simulink model "FMCW_Fixedpoint_model"  (R2025b)
settings: Solver=VariableStepAuto  StartTime=0.0  StopTime=10.0  RelTol=1e-3
libraries: phaseddetectlib x1, dspsrcs4 x1, dspxfrm3 x1, dspsigops x1, dspfdesign x1
settings Model: Creator=Yahin  LastModifiedBy=Yahin

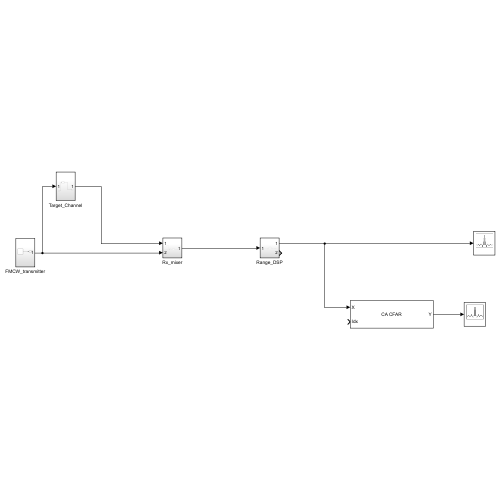
[thumbnail: Simulink's stored preview of the top-level diagram]
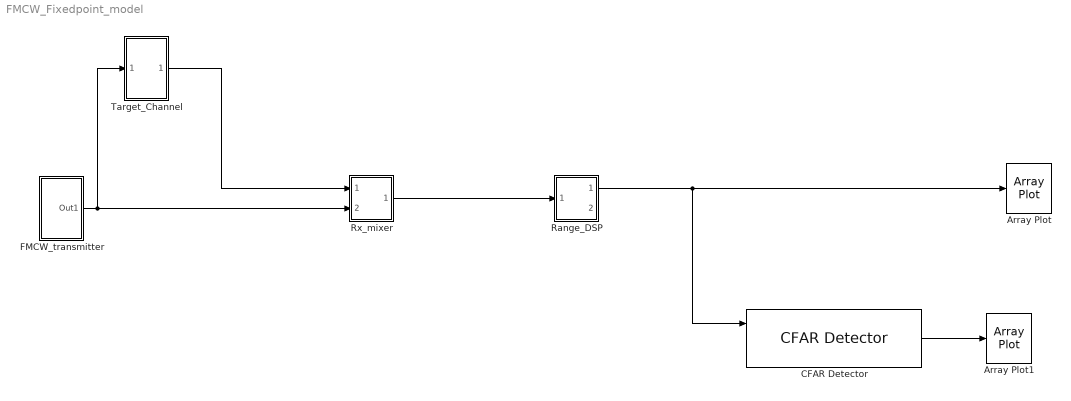
== system FMCW_Fixedpoint_model ==
  Array Plot : ArrayPlot  WindowPosition=[985.000000,385.000000,800.000000,500.000000,]  ScopeFrameLocation=window  YLimits=[-8.5215 76.8782]
  Array Plot1 : ArrayPlot  WindowPosition=[985.000000,385.000000,800.000000,500.000000,]  ScopeFrameLocation=window  YLimits=[-8.5215 76.8782]
  CFAR Detector : phaseddetectlib/CFAR Detector  Method=CA  Rank=1  NumGuardCells=4  NumTrainingCells=16  ThresholdFactor=Auto  ProbabilityFalseAlarm=1e-4  CustomThresholdFactor=1  OutputFormat=CUT result  ThresholdOutputPort=off  NoisePowerOutputPort=off  NumDetectionsSource=Auto  NumDetections=1  SimulateUsing=Interpreted execution
  FMCW_transmitter : Subsystem
  Range_DSP : Subsystem
  Rx_mixer : Subsystem
  Target_Channel : Subsystem
  wires:
  FMCW_transmitter/1(Out1) -> Rx_mixer/2(In2), Target_Channel/1(In1)
  Target_Channel/1(Out1) -> Rx_mixer/1(In1)
  Rx_mixer/1(Out1) -> Range_DSP/1(In1)
  Range_DSP/1(Out1) -> CFAR Detector/1, Array Plot/1
  CFAR Detector/1 -> Array Plot1/1

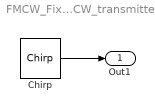
== system FMCW_Fixedpoint_model/FMCW_transmitter ==
  Chirp : dspsrcs4/Chirp  sweep=Linear  mode=Unidirectional  f0=0  f1=1000  t1=1  Tsweep=1  phase=0  Ts=1/2000  spf=1  datatype=double  OutputFrames=off
  Out1 : Outport
  wires:
  Chirp/1 -> Out1/1

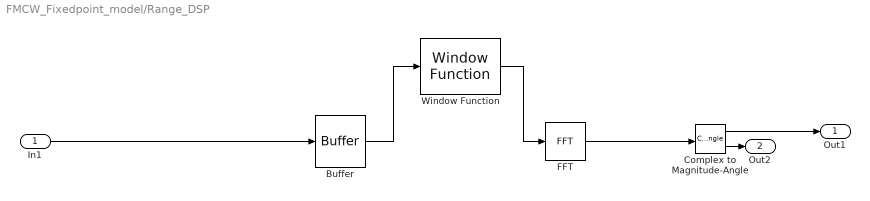
== system FMCW_Fixedpoint_model/Range_DSP ==
  In1 : Inport
  Buffer : Buffer  N=1024  OutputFrames=off
  Complex to Magnitude-Angle : ComplexToMagnitudeAngle
  FFT : dspxfrm3/FFT  FFTImplementation=Auto  CompMethod=Table lookup  TableOpt=NEW  TableOptActive=Speed  BitRevOrder=off  Normalize=off  InheritFFTLength=on  FFTLength=64  WrapInput=on  roundingMode=Ceiling  overflowMode=off  firstCoeffDataTypeStr=Inherit: Same word length as input  firstCoeffLastDataTypeStr=Inherit: Same word length as input  outputMin=[]  outputMax=[]
  Window Function : dspsigops/Window Function  winmode=Apply window to input  wintype=Hamming  sampmode=Continuous  samptime=1  N=64  Rs=50  beta=10  winsamp=Symmetric  UserWindow=hamming  OptParams=off  UserParams={'symmetric'}  dataType=double  isSigned=on  wordLen=16  udDataType=sfix(16)  fracBitsMode=Best precision  numFracBits=15  roundingMode=Floor  overflowMode=off  numSidelobes=4  sidelobeLevel=-30
  Out1 : Outport
  Out2 : Outport  Port=2
  wires:
  FFT/1 -> Complex to Magnitude-Angle/1
  Complex to Magnitude-Angle/2 -> Out2/1
  Window Function/1 -> FFT/1
  Buffer/1 -> Window Function/1
  Complex to Magnitude-Angle/1 -> Out1/1
  In1/1 -> Buffer/1

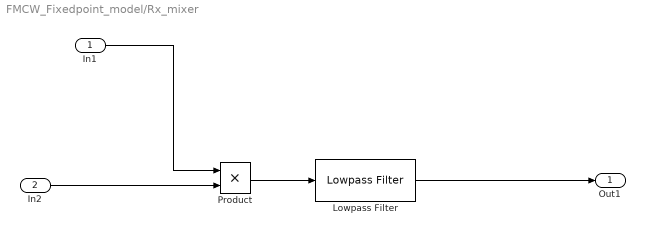
== system FMCW_Fixedpoint_model/Rx_mixer ==
  In1 : Inport
  In2 : Inport  Port=2
  Lowpass Filter : dspfdesign/Lowpass Filter  FilterType=FIR  DesignForMinimumOrder=on  FilterOrder=50  PassbandFrequency=1  StopbandFrequency=150  PassbandRipple=0.1  StopbandAttenuation=80  SampleRateMode=Specify on dialog  SampleRate=2000  SimulateUsing=Interpreted execution  roundingMode=Floor  coeffsDataTypeStr=fixdt(1,16)
  Product : Product
  Out1 : Outport
  wires:
  Product/1 -> Lowpass Filter/1
  In2/1 -> Product/2
  Lowpass Filter/1 -> Out1/1
  In1/1 -> Product/1

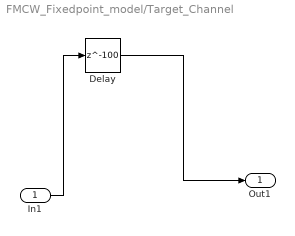
== system FMCW_Fixedpoint_model/Target_Channel ==
  In1 : Inport
  Delay : Delay  DelayLength=100
  Out1 : Outport
  wires:
  In1/1 -> Delay/1
  Delay/1 -> Out1/1
